simulink model "ideal_source_Motor_DVS_newest_param"  (R2025a)
settings: Solver=daessc  StartTime=0.0  StopTime=2  MaxStep=1e-7  RelTol=1e-3
model workspace (MAT data in the model file):
  FocDiscrTime = 0.0001
  Is_max = 390
  Ld = 0.0002
  Lq = 0.0002
  PolePairs = 13
  Psi = 0.07437
  Rs = 0.06
  compensate_pwm = 0
  piBandwidth = 5000
libraries: fl_lib x18, nesl_utility x15, mcbeeMathTransformLib x7, spsMeanLib x5, slpidlib x5, simulink x2, ee_lib x1, simulink_extras x1
(part 1 of 2)
settings Model: ParameterArgumentNames=FocDiscrTime,PolePairs,Psi  Creator=alexey  LastModifiedBy=alexey
settings SolverCC: ZeroCrossAlgorithm=Adaptive
settings OptimizationCC: DefaultParameterBehavior=Inlined  UseDivisionForNetSlopeComputation=on  GainParamInheritBuiltInType=on  UseFloatMulNetSlope=on  InlineInvariantSignals=on  ReuseModelBlockBuffer=off  EfficientFloat2IntCast=on  LifeSpan=1
settings DebuggingCC: IgnoredZcDiagnostic=none
settings HardwareCC: ProdLongLongMode=on
settings SFSimCC: MATLABDynamicMemAlloc=off
settings RTWCC: GenerateReport=on  LaunchReport=on  GPUComputeCapability=3.5
settings CodeAppCC: ForceParamTrailComments=on
settings GRTTargetCC: RTWCAPISignals=on  RTWCAPIParams=on  CombineSignalStateStructs=on  MatFileLogging=off  SupportVariableSizeSignals=on

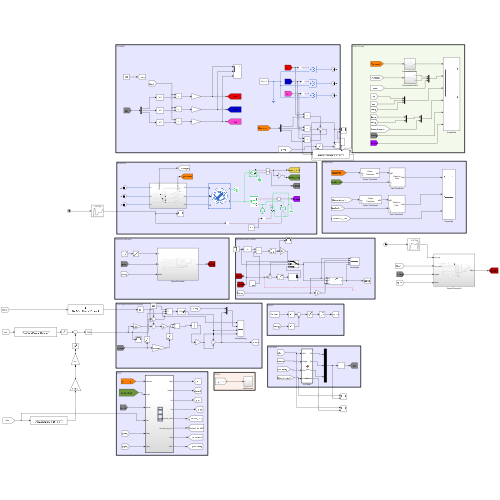
[thumbnail: Simulink's stored preview of the top-level diagram]
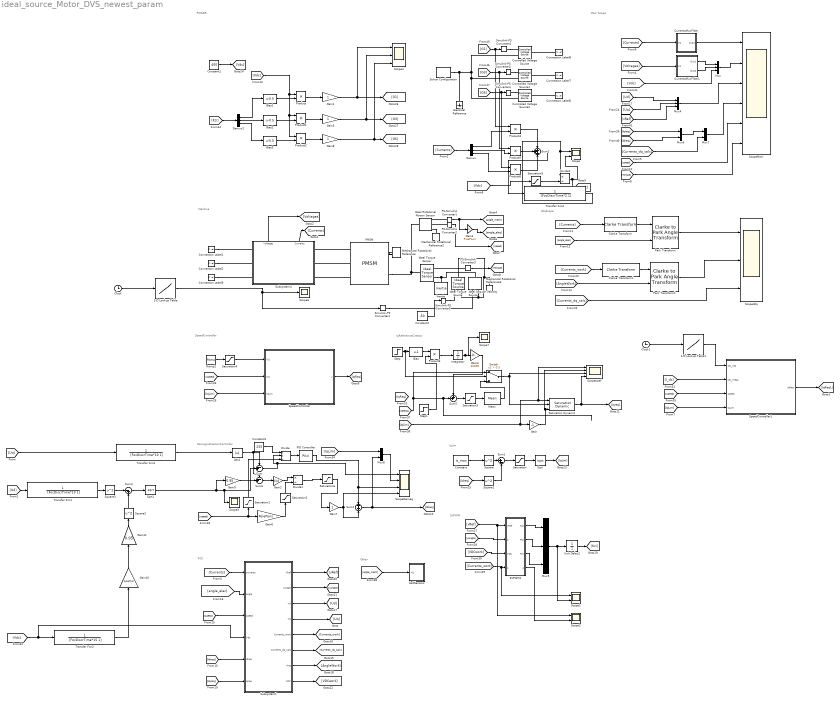
== system ideal_source_Motor_DVS_newest_param ==
  note: Main Scope
  note: POWER
  note: Other
  note: SVPWM
  note: FOC
  note: IqLim
  note: DemagnetizationController
  note: IdIqScope
  note: SpeedController
  note: IqReferenceCreator
  note: Machine
  1-D Lookup Table : Lookup_n-D  NumberOfTableDimensions=1  BreakpointsForDimension1=[0 0.2 0.3 0.45 0.7 1 1.5 1.6 1.7]  Table=[0 270 270 40 40 120 120 220 220]  InternalRulePriority=Speed  RndMeth=Simplest
  1-D Lookup Table1 : Lookup_n-D  NumberOfTableDimensions=1  BreakpointsForDimension1=[0 0.3 1 1.2 1.3 1.4 1.5]  Table=[0 200 150 200 30 250 250]  InternalRulePriority=Speed  RndMeth=Simplest
  Abs1 : Abs  SaturateOnIntegerOverflow=off
  Bias : Bias  Bias=-1  SaturateOnIntegerOverflow=off
  Bias1 : Bias  Bias=-0.5  SaturateOnIntegerOverflow=off
  Bias2 : Bias  Bias=-0.5  SaturateOnIntegerOverflow=off
  Bias3 : Bias  Bias=-0.5  SaturateOnIntegerOverflow=off
  Clarke Transform : mcbeeMathTransformLib/Clarke Transform  VariantControl=Variant2  PowerInvariant=off  UseWithEmbedded=on  PhaseInput=Three inputs
      settings: LibrarySourceBlock=mcbcontrolslib/Clarke Transform
  Clarke Transform1 : mcbeeMathTransformLib/Clarke Transform  VariantControl=Variant2  PowerInvariant=off  UseWithEmbedded=on  PhaseInput=Three inputs
      settings: LibrarySourceBlock=mcbcontrolslib/Clarke Transform
  Clock : Clock
  Clock1 : Clock
  Connection Label1 : ConnectionLabel  Label=A
  Connection Label2 : ConnectionLabel  Label=B
  Connection Label6 : ConnectionLabel  Label=C
  Connection Label7 : ConnectionLabel  Label=B
  Connection Label8 : ConnectionLabel  Label=A
  Connection Label9 : ConnectionLabel  Label=C
  Constant : Constant  Value=Is_max
  Constant1 : Constant  Value=400
  Constant2 : Constant  Value=-50
  Constant3 : Constant  Value=245
  Controlled Voltage Source : fl_lib/Electrical/Electrical Sources/Controlled Voltage Source
  Controlled Voltage Source1 : fl_lib/Electrical/Electrical Sources/Controlled Voltage Source
  Controlled Voltage Source2 : fl_lib/Electrical/Electrical Sources/Controlled Voltage Source
  CurrentsMuxFilter : Subsystem
  CurrentsMuxFilter1 : Subsystem
  Demux : Demux  Outputs=3
  Demux2 : Demux  Outputs=3
  Divide : Product  Inputs=**/
  Divide1 : Product  Inputs=*/
  Divide2 : Product  Inputs=*/
  Electrical Reference : fl_lib/Electrical/Electrical Elements/Electrical Reference
  Gain : Gain  Gain=-1
  Gain{1,5,7..8} (4 alike) : Gain
  Gain10 : Gain  Gain=1/sqrt(3)
  Gain11 : Gain  Gain=0.95
  Gain2 : Gain  Gain=1/Ld
  Gain3 : Gain  Gain=20000
  Gain4 : Gain  Gain=PolePairs
  Gain6 : Gain  Gain=PolePairs
  Gain9 : Gain  Gain=0.95
  HallSensors : Subsystem
  Ideal Angular Velocity Source : fl_lib/Mechanical/Mechanical Sources/Ideal Angular Velocity Source
  Ideal Rotational Motion Sensor : fl_lib/Mechanical/Mechanical Sensors/Ideal Rotational Motion Sensor  reference=foundation.enum.MeasurementReference.difference  acceleration_port=false  velocity_port=true  position_port=true  wrap_angle=false  offset=0 rad
  Ideal Torque Sensor : fl_lib/Mechanical/Mechanical Sensors/Ideal Torque Sensor
  Ideal Torque Source : fl_lib/Mechanical/Mechanical Sources/Ideal Torque Source
  Inertia : fl_lib/Mechanical/Rotational Elements/Inertia  inertia=0.1 kg*m^2  num_ports=foundation.enum.numPorts2.one  w_specify=off  w_priority=High  w=0 rad/s  w_nominal_specify=off  w_nominal_value=1  w_nominal_unit=rad/s  t_specify=off  t_priority=None  t=0 N*m  t_nominal_specify=off  t_nominal_value=1  t_nominal_unit=N*m
  Integrator : Integrator  LimitOutput=on  UpperSaturationLimit=0  LowerSaturationLimit=-2*Is_max/20000
  Mean : spsMeanLib/Mean  Freq=1000  Vinit=0  Ts=0
  Mechanical Rotational Reference : fl_lib/Mechanical/Rotational Elements/Mechanical Rotational Reference
  Mechanical Rotational Reference2 : fl_lib/Mechanical/Rotational Elements/Mechanical Rotational Reference
  Mechanical Rotational Reference3 : fl_lib/Mechanical/Rotational Elements/Mechanical Rotational Reference
  Mux : Mux  Inputs=3
  Mux4 : Mux  Inputs=3
  Mux5 : Mux  Inputs=3
  Mux6 : Mux  Inputs=2
  Mux7 : Mux  Inputs=2
  Mux8 : Mux  Inputs=2
  PID Controller : slpidlib/PID Controller  Controller=PI  Form=Parallel  TimeDomain=Discrete-time  UseExternalTs=off  SampleTime=FocDiscrTime  IntegratorMethod=Forward Euler  FilterMethod=Forward Euler  ControllerParametersSource=internal  P=0.1  I=500  UseKiTs=off  D=0.01  UseExternalDerivativeSource=off  N=100  UseFilter=on  TunerSelectOption=Transfer Function Based (PID Tuner App)  InitialConditionSource=internal  InitialConditionForIntegrator=0  InitialConditionForFilter=0  DifferentiatorICPrevScaledInput=0  ExternalReset=none  TrackingMode=off  Kt=1  LimitOutput=on  SatLimitsSource=internal  UpperSaturationLimit=0  LowerSaturationLimit=-250  LinearizeAsGain=on  AntiWindupMode=clamping  Kb=1  LimitIntegrator=off  UpperIntegratorSaturationLimit=inf  LowerIntegratorSaturationLimit=-inf  POutMin=[]  POutMax=[]  IOutMin=[]  IOutMax=[]  DOutMin=[]  DOutMax=[]  NOutMin=[]  NOutMax=[]  SumOutMin=[]  SumOutMax=[]  SaturationOutMin=[]  SaturationOutMax=[]  PParamMin=[]  PParamMax=[]  IParamMin=[]  IParamMax=[]  DParamMin=[]  DParamMax=[]  NParamMin=[]  NParamMax=[]  KbParamMin=[]  KbParamMax=[]  KtParamMin=[]  KtParamMax=[]  KbOutMin=[]  KbOutMax=[]  KtOutMin=[]  KtOutMax=[]  IntegratorOutMin=[]  IntegratorOutMax=[]  FilterOutMin=[]  FilterOutMax=[]  SumI1OutMin=[]  SumI1OutMax=[]  SumI2OutMin=[]  SumI2OutMax=[]  SumI3OutMin=[]  SumI3OutMax=[]  SumI4OutMin=[]  SumI4OutMax=[]  SumDOutMin=[]  SumDOutMax=[]  DifferentiatorOutMin=[]  DifferentiatorOutMax=[]  FilterDiffOutCoefMin=[]  FilterDiffOutCoefMax=[]  ReciprocalOutMin=[]  ReciprocalOutMax=[]  SumDenOutMin=[]  SumDenOutMax=[]  SumNumOutMin=[]  SumNumOutMax=[]  DivideOutMin=[]  DivideOutMax=[]  UdiffTsProdOutMin=[]  UdiffTsProdOutMax=[]  NTsProdOutMin=[]  NTsProdOutMax=[]  UintegralTsProdOutMin=[]  UintegralTsProdOutMax=[]  UngainTsProdOutMin=[]  UngainTsProdOutMax=[]  ClampingZeroOutDataTypeStr=Inherit: Inherit via back propagation  ClampingZeroOutMin=[]  ClampingZeroOutMax=[]  FilterDenConstantOutDataTypeStr=Inherit: Inherit via back propagation  FilterDenConstantOutMin=[]  FilterDenConstantOutMax=[]  PCopyOutDataTypeStr=Inherit: Inherit via back propagation  PCopyOutMin=[]  PCopyOutMax=[]  NCopyOutDataTypeStr=Inherit: Inherit via back propagation  NCopyOutMin=[]  NCopyOutMax=[]  IntegratorContinuousStateAttributes=''  IntegratorStateMustResolveToSignalObject=off  IntegratorRTWStateStorageClass=Auto  FilterContinuousStateAttributes=''  FilterStateMustResolveToSignalObject=off  FilterRTWStateStorageClass=Auto  ParallelPVariant=InternalParameters  IdealPVariant=Disabled  IVariant=InternalParameters  DVariant=Disabled  IntegratorVariant=Discrete  SatVariant=Enabled  AWVariant=DiscClampingParallel  PCopyVariant=Disabled  TRVariant=Disabled  FdbkBlocksVariant=Forward  IdealPFdbkVariant=Disabled  SatFdbkVariant=Disabled  DerivativeFilterVariant=Disabled  NVariant=Disabled  NCopyVariant=Disabled_SignalSpec  FilterICVariant=Disabled  IntegratorICVariant=InternalICs  ExternalResetVariant=Disabled  TRSumVariant=Passthrough  SumFdbkVariant=Disabled  SumVariant=Sum_PI  TsampFilterVariant=InternalTs  TsampNgainVariant=Passthrough  TsampIntegralVariant=Disabled_SignalSpec  ExternalSaturationOutDataTypeStr=Inherit: Same as second input  DerivativeSourceVariant=Disabled  PreIntVariant=InternalPreInt
  PMSM : ee_lib/Electromechanical/Permanent Magnet/PMSM  port_option=ee.enum.threePhasePort.expanded  winding_type=ee.enum.electromech.statorconfiguration.wye  machine_param=ee.enum.pmsm.parameterization.constant  nPolePairs=PolePairs  pmflux_param=ee.enum.pmflux.fluxlinkage  pm_flux_linkage=Psi Wb  torque_constant=0.074 N*m/A  back_emf_constant=0.06 V*s/rad  stator_param=ee.enum.statorparam.LdLqL0  Ld=Ld H  Lq=Lq H  idVec=[-200, 0, 200] A  iqVec=[-200, 0, 200] A  LdMatrix=0.0002 * ones(3, 3) H  LqMatrix=0.0002 * ones(3, 3) H  PmMatrix=0.1 * ones(3, 3) Wb  ktMatrix=0.18 * ones(3, 3) N*m/A  keMatrix=0.18 * ones(3, 3) V*s/rad  L0=1e-6 uH  Ls=0.0002 H  Lm=-0.00002 H  Ms=0.00002 H  Rs=Rs Ohm  zero_sequence=ee.enum.park.zerosequence.exclude  axes_param=ee.enum.rotorangle.daxis  loss_param=ee.enum.ironloss.none  losses_oc=[0, 0, 0] W  losses_sc=[0, 0, 0] W  f_losses=60 Hz  Isc_losses=95 A  J=0 kg*m^2  lam=0 N*m*s/rad  i_d_specify=on  i_d_priority=High  i_d=0 A  i_d_nominal_specify=off  i_d_nominal_value=1  i_d_nominal_unit=A  i_q_specify=on  i_q_priority=High  i_q=0 A  i_q_nominal_specify=off  i_q_nominal_value=1  i_q_nominal_unit=A  torque_specify=on  torque_priority=High  torque=0 N*m  torque_nominal_specify=off  torque_nominal_value=1  torque_nominal_unit=N*m  angular_velocity_specify=on  angular_velocity_priority=None  angular_velocity=7000 rpm  angular_velocity_nominal_specify=off  angular_velocity_nominal_value=1  angular_velocity_nominal_unit=rpm  angular_position_specify=on  angular_position_priority=High  angular_position=0 deg  angular_position_nominal_specify=off  angular_position_nominal_value=1  angular_position_nominal_unit=deg  alpha=3.93e-3 1/K  alpha_flux=-0.001 1/K  Tmeas=298.15 K  stator_thermal_mass=100 J/K  rotor_thermal_mass=200 J/K  Rm_percent_rotor=90  Rd_percent_rotor=30  temperatureA_specify=off  temperatureA_priority=High  temperatureA=25 degC  temperatureA_nominal_specify=off  temperatureA_nominal_value=1  temperatureA_nominal_unit=degC  temperatureB_specify=off  temperatureB_priority=High  temperatureB=25 degC  temperatureB_nominal_specify=off  temperatureB_nominal_value=1  temperatureB_nominal_unit=degC  temperatureC_specify=off  temperatureC_priority=High  temperatureC=25 degC  temperatureC_nominal_specify=off  temperatureC_nominal_value=1  temperatureC_nominal_unit=degC  temperatureR_specify=off  temperatureR_priority=High  temperatureR=25 degC  temperatureR_nominal_specify=off  temperatureR_nominal_value=1  temperatureR_nominal_unit=degC
      settings: InternalSimscapePortConfiguration="{\"Bottom\":[],\"Left\":[{\"id\":\"a\",\"label\":\"a\",\"type\":\"foundation.electrical.electrical\"},{\"id\":\"b\",\"label\":\"b\",\"type\":\"foundation.electrical.electrical\"},{\"id\":\"c\",\"label\":\"c\",\"type\":\"foundation.electrical.electrical\"}],\"Right\":[{\"id\":\"R\",\"label\":\"R\",\"type\":\"foundation.mechanical.rotational.rotational\"},{\"id\":\"C\",\"label\":\"C\",\"type\":\"foundation.mechanical.rotational.rotational\"}],\"Top\":[]}"
  PS-Simulink Converter1 : nesl_utility/PS-Simulink Converter  PhysicalDomain=network_engine_domain  SubClassName=ps_output  LeftPortType=input  RightPortType=output  PseudoPeriodic=off  Frequencies=[]  VectorFormat=inherit  Unit=inherit  AffineConversion=off
  PS-Simulink Converter2 : nesl_utility/PS-Simulink Converter  PhysicalDomain=network_engine_domain  SubClassName=ps_output  LeftPortType=input  RightPortType=output  PseudoPeriodic=off  Frequencies=[]  VectorFormat=inherit  Unit=inherit  AffineConversion=off
  PS-Simulink Converter3 : nesl_utility/PS-Simulink Converter  PhysicalDomain=network_engine_domain  SubClassName=ps_output  LeftPortType=input  RightPortType=output  PseudoPeriodic=off  Frequencies=[]  VectorFormat=inherit  Unit=inherit  AffineConversion=off
  Park Transform : mcbeeMathTransformLib/Clarke to Park Angle Transform  AxisAlignment=D-axis  UseWithEmbedded=on  PhaseInput=Three inputs  ThetaInput=Electrical position  AngleInput=Radians  N_points=1024
      settings: LibrarySourceBlock=mcbcontrolslib/Park Transform
  Park Transform1 : mcbeeMathTransformLib/Clarke to Park Angle Transform  AxisAlignment=D-axis  UseWithEmbedded=on  PhaseInput=Three inputs  ThetaInput=Electrical position  AngleInput=Radians  N_points=1024
      settings: LibrarySourceBlock=mcbcontrolslib/Park Transform
  Product{,1..6} (7 alike) : Product
  Ramp2 : simulink/Sources/Ramp  slope=300/4e-3  start=1e-3  InitialOutput=0
  SVPWM1 : MATLAB Function  TreatAsAtomicUnit=on  SystemSampleTime=FocDiscrTime/2
  Saturation : Saturate  UpperLimit=inf  LowerLimit=0
  Saturation Dynamic : simulink/Discontinuities/Saturation Dynamic  OutMin=[]  OutMax=[]  OutDataTypeStr=Inherit: Same as second input  OutDataType=fixdt(1, 16)  OutScaling=2^-10  DoSatur=off
  Saturation1 : Saturate  UpperLimit=inf  LowerLimit=1
  Saturation2 : Saturate  UpperLimit=inf  LowerLimit=1
  Saturation3 : Saturate  UpperLimit=inf  LowerLimit=-Is_max
  Saturation4 : Saturate  UpperLimit=600  LowerLimit=0
  Saturation5 : Saturate  UpperLimit=inf  LowerLimit=1
  Saturation6 : Saturate  UpperLimit=0  LowerLimit=-100
  Scope : Scope  NumInputPorts=2
      settings: ActiveDisplayYMinimum=-51831.017888207687  ActiveDisplayYMaximum=5759.0019876081242  DataLoggingVariableName=ScopeData8
  Scope1 : Scope  NumInputPorts=2
      settings: ActiveDisplayYMinimum=-438.55416313604536  ActiveDisplayYMaximum=438.95198817062709
  Scope2 : Scope  NumInputPorts=2
      settings: ActiveDisplayYMinimum=192.19580526011231  ActiveDisplayYMaximum=251.38218785320146  DataLoggingVariableName=ScopeData2
  Scope3 : Scope
      settings: ActiveDisplayYMinimum=58.599899423791321  ActiveDisplayYMaximum=245.7111222862454  DataLoggingVariableName=ScopeData12
  Scope4 : Scope  NumInputPorts=3
      settings: ActiveDisplayYMinimum=-300  ActiveDisplayYMaximum=-100  DataLoggingVariableName=ScopeData14
  Scope6 : Scope
      settings: ActiveDisplayYMinimum=-68.247393749999986  ActiveDisplayYMaximum=614.22654375  DataLoggingVariableName=ScopeData15
  Scope7 : Scope
      settings: DataLoggingVariableName=ScopeData16
  ScopeDemag : Scope  NumInputPorts=4
      settings: ActiveDisplayYMinimum=100.15963791243919  ActiveDisplayYMaximum=100.26275452875461  DataLoggingVariableName=ScopeData7
  ScopeIdIq : Scope  NumInputPorts=3
      settings: ActiveDisplayYMinimum=-200.18878641188479  ActiveDisplayYMaximum=389.61354814376449  DataLoggingVariableName=ScopeData13
  ScopeIqref : Scope  NumInputPorts=4
      settings: ActiveDisplayYMinimum=300.59489839356036  ActiveDisplayYMaximum=316.60056684515996  DataLoggingVariableName=ScopeData11
  ScopeMain : Scope  NumInputPorts=6
      settings: ActiveDisplayYMinimum=-484.90618085327424  ActiveDisplayYMaximum=498.32290898369712  DataLoggingVariableName=ScopeData9
  Simulink-PS Converter1 : nesl_utility/Simulink-PS Converter  PhysicalDomain=network_engine_domain  SubClassName=ps_input  LeftPortType=input  RightPortType=output  PseudoPeriodic=off  Frequencies=[]  NoiseDistribution=none  NoiseParameters=[]  Unit=1  AffineConversion=off  FilteringAndDerivatives=filter  SimscapeFilterOrder=1  InputFilterTimeConstant=1e-3  UdotUserProvided=0
  Simulink-PS Converter2 : nesl_utility/Simulink-PS Converter  PhysicalDomain=network_engine_domain  SubClassName=ps_input  LeftPortType=input  RightPortType=output  PseudoPeriodic=off  Frequencies=[]  NoiseDistribution=none  NoiseParameters=[]  Unit=1  AffineConversion=off  FilteringAndDerivatives=provide  SimscapeFilterOrder=1  InputFilterTimeConstant=0.001  UdotUserProvided=0
  Simulink-PS Converter3 : nesl_utility/Simulink-PS Converter  PhysicalDomain=network_engine_domain  SubClassName=ps_input  LeftPortType=input  RightPortType=output  PseudoPeriodic=off  Frequencies=[]  NoiseDistribution=none  NoiseParameters=[]  Unit=1  AffineConversion=off  FilteringAndDerivatives=provide  SimscapeFilterOrder=1  InputFilterTimeConstant=0.001  UdotUserProvided=0
  Simulink-PS Converter4 : nesl_utility/Simulink-PS Converter  PhysicalDomain=network_engine_domain  SubClassName=ps_input  LeftPortType=input  RightPortType=output  PseudoPeriodic=off  Frequencies=[]  NoiseDistribution=none  NoiseParameters=[]  Unit=1  AffineConversion=off  FilteringAndDerivatives=provide  SimscapeFilterOrder=1  InputFilterTimeConstant=0.001  UdotUserProvided=0
  Simulink-PS Converter5 : nesl_utility/Simulink-PS Converter  PhysicalDomain=network_engine_domain  SubClassName=ps_input  LeftPortType=input  RightPortType=output  PseudoPeriodic=off  Frequencies=[]  NoiseDistribution=none  NoiseParameters=[]  Unit=1  AffineConversion=off  FilteringAndDerivatives=filter  SimscapeFilterOrder=1  InputFilterTimeConstant=1e-3  UdotUserProvided=0
  Solver Configuration : nesl_utility/Solver Configuration  PhysicalDomain=network_engine_domain  SubClassName=solver  LeftPortType=input  RightPortType=generic  Tones=[]  Harmonics=[]  SimulateNoise=off  Profile=off  UseLocalSampling=off  EnableSwitchedLinearOptims=on  FrequencyDomain=off  UseCCode=off  RelTol=0.001  AbsTol=0.001  MinStep=1e-09  ToWorkspace=off  RevertToSquareIcSolve=off  NumHomotopyIterations=100  PhasorMode=off  PhasorModeNumHarmonics=1  ConsistencySolver=NEWTON_XTOL_AFTER_FTOL  IndexReductionMethod=DerivativeReplacement  DoDC=off  ResidualTolerance=1e-09  ConsistencyTolSource=GLOBAL  ConsistencyAbsTol=0.001  ConsistencyRelTol=0.001  ConsistencyTolFactor=0.001  UseLocalSolver=off  LocalSolverChoice=NE_BACKWARD_EULER_ADVANCER  ResolveIndetEquations=on  FunctionEvalNumThread=1  LocalSolverSampleTime=0.001  DoFixedCost=off  MaxNonlinIter=3  MaxModeIter=2  ComputeImpulses=off  ImpulseIterations=2  LinearAlgebra=auto  LinearAlgebraNumThread=0  EquationFormulation=NE_TIME_EF  DelaysMemoryBudget=1024  AutomaticFiltering=on  FilteringTimeConstant=0.001  PartitionStorageMethod=AS_NEEDED  PartitionMemoryBudget=1024  PartitionMethod=ROBUST  MultibodyUseLocalSolver=off  MultibodyLocalSolverChoice=ODE1  MultibodyLocalSolverSampleTime=0.001
  SpeedController : Subsystem
  SpeedController1 : Subsystem
  Sqrt : Sqrt
  Sqrt1 : Sqrt
  Square{,1..3} (4 alike) : Math  Operator=square
  Step : Step  Time=2  Before=1  After=0  SampleTime=0
  Step1 : Step  Time=0.7  Before=1  After=-1  SampleTime=0
  Subsystem1 : Subsystem  TreatAsAtomicUnit=on  SystemSampleTime=FocDiscrTime
  Subsystem4 : Subsystem
      settings: PortSchema="{\"entries\":[{\"content\":{\"sides\":[{\"content\":{},\"type\":\"ConnectorPlacement.EquallySpacedRectSide\",\"uuid\":\"18ff9a98-da5f-4d42-bf88-8b80acaefaab\"},{\"content\":{\"connectorIds\":[\"Out1\",\"Out2\"],\"side\":\"RIGHT\"},\"type\":\"ConnectorPlacement.EquallySpacedRectSide\",\"uuid\":\"2ae2e449-c022-4e43-8d74-e7903f555369\"},{\"content\":{\"connectorIds\":[\"LConn1\",\"LConn2\",\"LConn3\"],\"side\":\"TOP\"},\"type\":\"ConnectorPlacement.EquallySpacedRectSide\",\"uuid\":\"55b123c9-903d-428f-ba92-02a5913ccae5\"},{\"content\":{\"connectorIds\":[\"RConn1\",\"RConn2\",\"RConn3\"],\"side\":\"BOTTOM\"},\"type\":\"ConnectorPlacement.EquallySpacedRectSide\",\"uuid\":\"b028b0af-4fd3-4535-8d3b-f50dc0cabb29\"}]},\"type\":\"ConnectorPlacement.EquallySpacedConnector\",\"uuid\":\"08d0fd08-360e-4301-974e-a78b2c2bf0b9\"}],\"packageUris\":[\"http://schema.mathworks.com/mf0/Connector/R2020b\"],\"version\":\"1.0\"}"
  Sum : Sum  Inputs=-+|
  Sum1 : Sum  Inputs=|+-
  Sum2 : Sum  Inputs=+++
  Sum3 : Sum  Inputs=|-+
  Sum4 : Sum
  Sum5 : Sum  Inputs=++|
  Sum6 : Sum  Inputs=-+|
  Switch : Switch  Criteria=u2 > Threshold  Threshold=0.5  SaturateOnIntegerOverflow=off  InputSameDT=off
  Transfer Fcn1 : TransferFcn  Denominator=[FocDiscrTime*10 1]
  Transfer Fcn2 : TransferFcn  Denominator=[FocDiscrTime*15 1]
  Transfer Fcn3 : TransferFcn  Denominator=[FocDiscrTime*10 1]
  Transfer Fcn4 : TransferFcn  Denominator=[FocDiscrTime*2 1]
  Unit Delay2 : UnitDelay  SampleTime=FocDiscrTime/2  HasFrameUpgradeWarning=on
  wires:
  CurrentsMuxFilter/1(Out2) -> ScopeMain/1
  [Currents] -> CurrentsMuxFilter/1(In1)
  Mux/1 -> ScopeMain/2
  CurrentsMuxFilter1/1(Out1) -> Mux/1
  [Torque] -> ScopeMain/6
  [speed] -> ScopeMain/5
  [Vdc] -> Mux/3
  CurrentsMuxFilter1/2(Out2) -> Mux/2
  [Voltages] -> CurrentsMuxFilter1/1(In1)
  [Ud] -> Mux4/1
  [Uq] -> Mux4/2
  Mux4/1 -> ScopeMain/3
  [Currents_dq_calc] -> Mux7/2
  [Idreq] -> Mux6/2
  [Iqreq] -> Mux6/1
  Mux6/1 -> Mux7/1
  Mux7/1 -> ScopeMain/4
  [vRef] -> Mux4/3
  Gain8/1 -> [G5], Scope4/3
  Gain5/1 -> [G3], Scope4/2
  Gain1/1 -> [G1], Scope4/1
  [Vdc] -> Product/1, Product1/1, Product2/1
  Product2/1 -> Gain8/1
  Product1/1 -> Gain5/1
  Product/1 -> Gain1/1
  Bias3/1 -> Product2/2
  Bias2/1 -> Product1/2
  Bias1/1 -> Product/2
  [G3] -> Product5/1, Simulink-PS Converter3/1
  [G5] -> Product6/1, Simulink-PS Converter4/1
  [G1] -> Product4/1, Simulink-PS Converter2/1
  Demux2/3 -> Bias3/1
  Demux2/2 -> Bias2/1
  Demux2/1 -> Bias1/1
  [Kzi] -> Demux2/1
  Saturation1/1 -> Divide/3
  Constant3/1 -> Divide/1
  Divide/1 -> PID Controller/1
  Gain11/1 -> Square2/1
  Saturation6/1 -> Gain7/1
  Gain2/1 -> Divide1/1
  Transfer Fcn3/1 -> Abs1/1
  Divide1/1 -> Saturation6/1
  Gain9/1 -> Sum6/2
  Gain7/1 -> ScopeDemag/4, Sum4/2
  Sum6/1 -> Gain2/1
  Mux8/1 -> ScopeDemag/2
  Transfer Fcn2/1 -> Gain10/1
  Abs1/1 -> Sum/1, Sum6/1
  Sum/1 -> ScopeDemag/1, Divide/2
  Clock/1 -> 1-D Lookup Table/1
  Constant2/1 -> Simulink-PS Converter5/1
  [Idreq] -> Square1/1
  [IqReq1] -> Switch/1, Sum5/2
  Saturation3/1 -> Mean/1
  Gain3/1 -> Sum5/1
  Sum5/1 -> Saturation3/1
  Mean/1 -> Switch/3
  Integrator/1 -> Gain3/1, Scope7/1
  Product3/1 -> Integrator/1
  Saturation Dynamic/1 -> [Iqreq], ScopeIqref/4
  Switch/1 -> Saturation Dynamic/2, ScopeIqref/3
  [IqLim] -> Gain/1, ScopeIqref/1, Saturation Dynamic/1
  Gain/1 -> ScopeIqref/2, Saturation Dynamic/3
  Step1/1 -> Product3/2
  Step/1 -> Switch/2, Bias/1
  Bias/1 -> Product3/1
  1-D Lookup Table/1 -> Scope6/1, Simulink-PS Converter1/1
  [Ud] -> Transfer Fcn1/1
  Sum3/1 -> Sqrt1/1
  Square3/1 -> Sum3/1
  Transfer Fcn1/1 -> Square3/1
  Gain10/1 -> Gain11/1
  Square2/1 -> Sum3/2
  Sqrt1/1 -> Sum/2, Scope3/1, Gain9/1
  SVPWM1/4(vRefwork) -> Scope2/2
  [Uq] -> Transfer Fcn3/1
  [angle_mech] -> HallSensors/1(In1)
  PID Controller/1 -> ScopeDemag/3, Sum4/1
  Gain6/1 -> Saturation2/1
  [IqLim] -> Mux8/1
  [IqLim] -> SpeedController/3(IqLim)
  SVPWM1/3(Tct) -> Mux5/3
  SVPWM1/2(Tbt) -> Mux5/2
  SVPWM1/1(Tat) -> Mux5/1
  [VDCwork] -> SVPWM1/3(VDC)
  [vAngle] -> SVPWM1/2(vAngle)
  [Currents_work] -> SVPWM1/4(Currents), Scope1/1
  [vRef] -> SVPWM1/1(vRef), Scope2/1
  Subsystem1/1(vRef) -> [vRef]
  Subsystem1/8(VDC) -> [VDCwork]
  Subsystem1/2(vAngle) -> [vAngle]
  Unit Delay2/1 -> [Kzi]
  Mux5/1 -> Unit Delay2/1, Scope1/2
  Subsystem1/7(Ang) -> [AngleWork]
  Subsystem1/3(Vd) -> [Ud]
  [Currents_work] -> Clarke Transform1/1
  Clarke Transform1/1 -> Park Transform1/1
  [AngleWork] -> Park Transform1/2
  Park Transform1/1 -> ScopeIdIq/2
  Subsystem1/6(Currents_dq_calc) -> [Currents_dq_calc]
  Subsystem1/5(Currents_work) -> [Currents_work]
  Saturation4/1 -> SpeedController/1(In1)
  [Iqreq] -> Subsystem1/6(Iqreq)
  [Idreq] -> Subsystem1/5(Idreq)
  Subsystem1/4(Vq) -> [Uq]
  SpeedController/1(y) -> [IqReq]
  [speed] -> SpeedController/2(In2)
  Ramp2/1 -> Saturation4/1
  [speed] -> Gain6/1, Saturation1/1
  [Currents_dq_calc] -> ScopeIdIq/3
  Park Transform/1 -> ScopeIdIq/1
  [angle_elec] -> Park Transform/2
  Clarke Transform/1 -> Park Transform/1
  [Currents] -> Clarke Transform/1
  PS-Simulink Converter1/1 -> [angle_mech], Gain4/1
  Gain4/1 -> [angle_elec]
  [speed] -> Subsystem1/3(speed)
  Subsystem4/2(Currents) -> [Currents]
  Square1/1 -> Sum1/2
  Sum4/1 -> Mux8/2, [Idreq]
  Square/1 -> Sum1/1
  PS-Simulink Converter2/1 -> [speed]
  [Currents] -> Subsystem1/1(currents)
  Sum1/1 -> Saturation/1
  Saturation/1 -> Sqrt/1
  PS-Simulink Converter3/1 -> [Torque]
  Sqrt/1 -> [IqLim]
  Constant/1 -> Square/1
  Subsystem4/1(Voltages) -> [Voltages]
  [angle_elec] -> Subsystem1/2(angle)
  Saturation2/1 -> Divide1/2
  Constant1/1 -> [Vdc]
  [Vdc] -> Subsystem1/4(Vdc), Transfer Fcn2/1
  [Currents] -> Demux/1
  Demux/1 -> Product4/2
  Demux/2 -> Product5/2
  Demux/3 -> Product6/2
  Product4/1 -> Sum2/1
  Product5/1 -> Sum2/2
  Product6/1 -> Sum2/3
  Sum2/1 -> Transfer Fcn4/1
  [Vdc] -> Saturation5/1
  Divide2/1 -> [I_dc], Scope/2
  Saturation5/1 -> Divide2/2
  Transfer Fcn4/1 -> Divide2/1, Scope/1
  Clock1/1 -> 1-D Lookup Table1/1
  [speed] -> SpeedController1/3(speed)
  SpeedController1/1(IqReq) -> [IqReq1]
  [I_dc] -> SpeedController1/2(Idc_meas)
  1-D Lookup Table1/1 -> SpeedController1/1(Idc_req)
  [IqLim] -> SpeedController1/4(IqLim)
  connections:
  Solver Configuration/RConn1 -- Electrical Reference/LConn1 -- Controlled Voltage Source/RConn2 -- Controlled Voltage Source2/RConn2 -- Controlled Voltage Source1/RConn2
  Simulink-PS Converter3/RConn1 -- Controlled Voltage Source1/RConn1
  Connection Label7/LConn1 -- Controlled Voltage Source1/LConn1
  Simulink-PS Converter2/RConn1 -- Controlled Voltage Source/RConn1
  Connection Label8/LConn1 -- Controlled Voltage Source/LConn1
  Connection Label6/LConn1 -- Controlled Voltage Source2/LConn1
  Simulink-PS Converter4/RConn1 -- Controlled Voltage Source2/RConn1
  Ideal Torque Sensor/LConn1 -- Ideal Rotational Motion Sensor/LConn1 -- PMSM/RConn1
  Mechanical Rotational Reference3/LConn1 -- Ideal Torque Source/RConn2 -- Ideal Angular Velocity Source/RConn2 -- Ideal Torque Source/LConn1
  Ideal Torque Sensor/RConn1 -- Inertia/LConn1 -- Ideal Angular Velocity Source/LConn1
  PS-Simulink Converter2/LConn1 -- Ideal Rotational Motion Sensor/RConn2
  PMSM/RConn2 -- Mechanical Rotational Reference/LConn1
  Connection Label1/LConn1 -- Subsystem4/LConn3
  PMSM/LConn2 -- Subsystem4/RConn2
  PS-Simulink Converter3/LConn1 -- Ideal Torque Sensor/RConn2
  Simulink-PS Converter1/RConn1 -- Ideal Angular Velocity Source/RConn1
  Connection Label9/LConn1 -- Subsystem4/LConn1
  Connection Label2/LConn1 -- Subsystem4/LConn2
  PMSM/LConn3 -- Subsystem4/RConn3
  PS-Simulink Converter1/LConn1 -- Ideal Rotational Motion Sensor/RConn3
  PMSM/LConn1 -- Subsystem4/RConn1
  Ideal Rotational Motion Sensor/RConn1 -- Mechanical Rotational Reference2/LConn1
  Simulink-PS Converter5/RConn1 -- Ideal Torque Source/RConn1

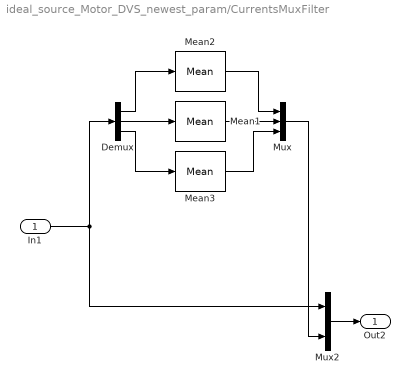
== system ideal_source_Motor_DVS_newest_param/CurrentsMuxFilter ==
  In1 : Inport
  Demux : Demux  Outputs=3
  Mean1 : spsMeanLib/Mean  Freq=20000  Vinit=0  Ts=0
  Mean2 : spsMeanLib/Mean  Freq=20000  Vinit=0  Ts=0
  Mean3 : spsMeanLib/Mean  Freq=20000  Vinit=0  Ts=0
  Mux : Mux  Inputs=3
  Mux2 : Mux  Inputs=2
  Out2 : Outport
  wires:
  Mean3/1 -> Mux/3
  Mean1/1 -> Mux/2
  Mean2/1 -> Mux/1
  Demux/3 -> Mean3/1
  Demux/2 -> Mean1/1
  Demux/1 -> Mean2/1
  Mux2/1 -> Out2/1
  In1/1 -> Mux2/1, Demux/1
  Mux/1 -> Mux2/2

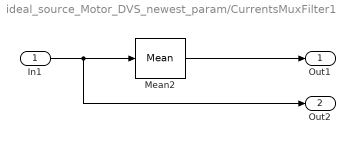
== system ideal_source_Motor_DVS_newest_param/CurrentsMuxFilter1 ==
  In1 : Inport
  Mean2 : spsMeanLib/Mean  Freq=20000  Vinit=0  Ts=0
  Out1 : Outport
  Out2 : Outport  Port=2
  wires:
  In1/1 -> Mean2/1, Out2/1
  Mean2/1 -> Out1/1

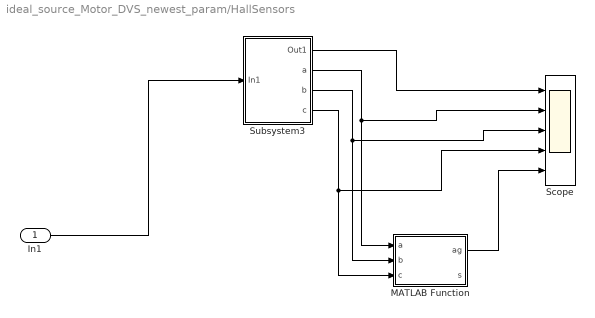
== system ideal_source_Motor_DVS_newest_param/HallSensors ==
  In1 : Inport
  MATLAB Function : MATLAB Function  TreatAsAtomicUnit=on  SystemSampleTime=1/40000
  Scope : Scope  NumInputPorts=5
      settings: ActiveDisplayYMinimum=-0.7854  ActiveDisplayYMaximum=7.06858  DataLoggingVariableName=ScopeData3
  Subsystem3 : Subsystem
  wires:
  Subsystem3/1(Out1) -> Scope/1
  Subsystem3/4(c) -> Scope/4, MATLAB Function/3(c)
  Subsystem3/2("a ") -> Scope/2, MATLAB Function/1(a)
  MATLAB Function/1(ag) -> Scope/5
  Subsystem3/3(b) -> Scope/3, MATLAB Function/2(b)
  In1/1 -> Subsystem3/1(In1)

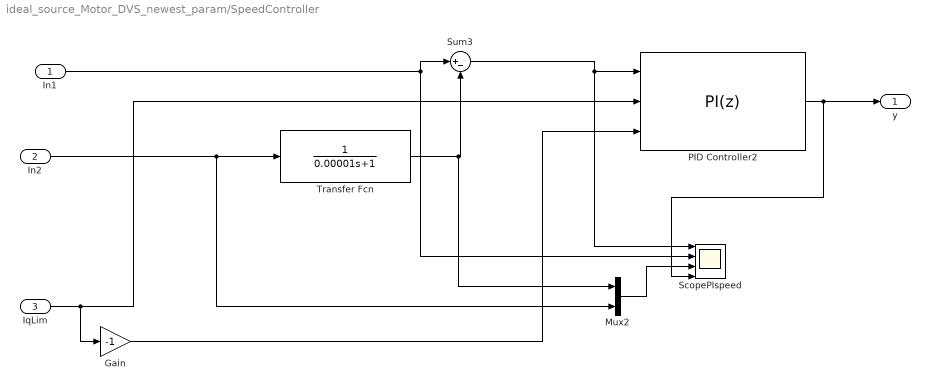
== system ideal_source_Motor_DVS_newest_param/SpeedController ==
  In1 : Inport
  In2 : Inport  Port=2
  IqLim : Inport  Port=3
  Gain : Gain  Gain=-1
  Mux2 : Mux  Inputs=2
  PID Controller2 : slpidlib/PID Controller  Controller=PI  Form=Parallel  TimeDomain=Discrete-time  UseExternalTs=off  SampleTime=FocDiscrTime  IntegratorMethod=Forward Euler  FilterMethod=Forward Euler  ControllerParametersSource=internal  P=5  I=1  UseKiTs=off  D=0  UseExternalDerivativeSource=off  N=100  UseFilter=on  TunerSelectOption=Transfer Function Based (PID Tuner App)  InitialConditionSource=internal  InitialConditionForIntegrator=0  InitialConditionForFilter=0  DifferentiatorICPrevScaledInput=0  ExternalReset=none  TrackingMode=off  Kt=1  LimitOutput=on  SatLimitsSource=external  UpperSaturationLimit=350  LowerSaturationLimit=-3  LinearizeAsGain=on  AntiWindupMode=clamping  Kb=1  LimitIntegrator=off  UpperIntegratorSaturationLimit=inf  LowerIntegratorSaturationLimit=-inf  POutMin=[]  POutMax=[]  IOutMin=[]  IOutMax=[]  DOutMin=[]  DOutMax=[]  NOutMin=[]  NOutMax=[]  SumOutMin=[]  SumOutMax=[]  SaturationOutMin=[]  SaturationOutMax=[]  PParamMin=[]  PParamMax=[]  IParamMin=[]  IParamMax=[]  DParamMin=[]  DParamMax=[]  NParamMin=[]  NParamMax=[]  KbParamMin=[]  KbParamMax=[]  KtParamMin=[]  KtParamMax=[]  KbOutMin=[]  KbOutMax=[]  KtOutMin=[]  KtOutMax=[]  IntegratorOutMin=[]  IntegratorOutMax=[]  FilterOutMin=[]  FilterOutMax=[]  SumI1OutMin=[]  SumI1OutMax=[]  SumI2OutMin=[]  SumI2OutMax=[]  SumI3OutMin=[]  SumI3OutMax=[]  SumI4OutMin=[]  SumI4OutMax=[]  SumDOutMin=[]  SumDOutMax=[]  DifferentiatorOutMin=[]  DifferentiatorOutMax=[]  FilterDiffOutCoefMin=[]  FilterDiffOutCoefMax=[]  ReciprocalOutMin=[]  ReciprocalOutMax=[]  SumDenOutMin=[]  SumDenOutMax=[]  SumNumOutMin=[]  SumNumOutMax=[]  DivideOutMin=[]  DivideOutMax=[]  UdiffTsProdOutMin=[]  UdiffTsProdOutMax=[]  NTsProdOutMin=[]  NTsProdOutMax=[]  UintegralTsProdOutMin=[]  UintegralTsProdOutMax=[]  UngainTsProdOutMin=[]  UngainTsProdOutMax=[]  ClampingZeroOutDataTypeStr=Inherit: Inherit via back propagation  ClampingZeroOutMin=[]  ClampingZeroOutMax=[]  FilterDenConstantOutDataTypeStr=Inherit: Inherit via back propagation  FilterDenConstantOutMin=[]  FilterDenConstantOutMax=[]  PCopyOutDataTypeStr=Inherit: Inherit via back propagation  PCopyOutMin=[]  PCopyOutMax=[]  NCopyOutDataTypeStr=Inherit: Inherit via back propagation  NCopyOutMin=[]  NCopyOutMax=[]  IntegratorContinuousStateAttributes=''  IntegratorStateMustResolveToSignalObject=off  IntegratorRTWStateStorageClass=Auto  FilterContinuousStateAttributes=''  FilterStateMustResolveToSignalObject=off  FilterRTWStateStorageClass=Auto  ParallelPVariant=InternalParameters  IdealPVariant=Disabled  IVariant=InternalParameters  DVariant=Disabled  IntegratorVariant=Discrete  SatVariant=External  AWVariant=DiscClampingParallel  PCopyVariant=Disabled  TRVariant=Disabled  FdbkBlocksVariant=Forward  IdealPFdbkVariant=Disabled  SatFdbkVariant=Disabled  DerivativeFilterVariant=Disabled  NVariant=Disabled  NCopyVariant=Disabled_SignalSpec  FilterICVariant=Disabled  IntegratorICVariant=InternalICs  ExternalResetVariant=Disabled  TRSumVariant=Passthrough  SumFdbkVariant=Disabled  SumVariant=Sum_PI  TsampFilterVariant=InternalTs  TsampNgainVariant=Passthrough  TsampIntegralVariant=Disabled_SignalSpec  ExternalSaturationOutDataTypeStr=Inherit: Same as second input  DerivativeSourceVariant=Disabled  PreIntVariant=InternalPreInt
  ScopePIspeed : Scope  NumInputPorts=4
      settings: ActiveDisplayYMinimum=-74.200839679499552  ActiveDisplayYMaximum=662.92601742403372  DataLoggingVariableName=ScopeData10
  Sum3 : Sum  Inputs=|+-
  Transfer Fcn : TransferFcn  Denominator=[0.00001 1]
  y : Outport
  wires:
  Gain/1 -> PID Controller2/3
  IqLim/1 -> PID Controller2/2, Gain/1
  In1/1 -> ScopePIspeed/2, Sum3/1
  Transfer Fcn/1 -> Sum3/2, Mux2/1
  Sum3/1 -> PID Controller2/1, ScopePIspeed/1
  PID Controller2/1 -> ScopePIspeed/4, y/1
  In2/1 -> Transfer Fcn/1, Mux2/2
  Mux2/1 -> ScopePIspeed/3

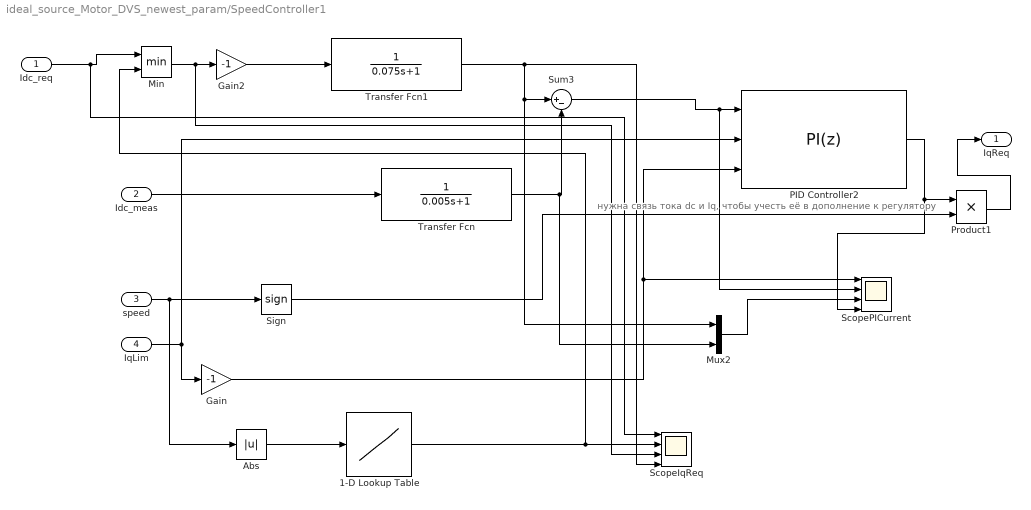
== system ideal_source_Motor_DVS_newest_param/SpeedController1 ==
  note: нужна связь тока dc и Iq, чтобы учесть её в дополнение к регулятору
  Idc_req : Inport
  Idc_meas : Inport  Port=2
  speed : Inport  Port=3
  IqLim : Inport  Port=4
  1-D Lookup Table : Lookup_n-D  NumberOfTableDimensions=1  BreakpointsForDimension1=[0 550 600 1200 1925 2350 2400 2450]*0.1047  Table=[0 0 69 115 115 50 0 0]  InternalRulePriority=Speed  RndMeth=Simplest
  Abs : Abs  SaturateOnIntegerOverflow=off
  Gain : Gain  Gain=-1
  Gain2 : Gain  Gain=-1
  Min : MinMax  Inputs=2
  Mux2 : Mux  Inputs=2
  PID Controller2 : slpidlib/PID Controller  Controller=PI  Form=Parallel  TimeDomain=Discrete-time  UseExternalTs=off  SampleTime=FocDiscrTime  IntegratorMethod=Forward Euler  FilterMethod=Forward Euler  ControllerParametersSource=internal  P=5  I=450  UseKiTs=off  D=0  UseExternalDerivativeSource=off  N=100  UseFilter=on  TunerSelectOption=Transfer Function Based (PID Tuner App)  InitialConditionSource=internal  InitialConditionForIntegrator=0  InitialConditionForFilter=0  DifferentiatorICPrevScaledInput=0  ExternalReset=none  TrackingMode=off  Kt=1  LimitOutput=on  SatLimitsSource=external  UpperSaturationLimit=350  LowerSaturationLimit=-3  LinearizeAsGain=on  AntiWindupMode=clamping  Kb=1  LimitIntegrator=off  UpperIntegratorSaturationLimit=inf  LowerIntegratorSaturationLimit=-inf  POutMin=[]  POutMax=[]  IOutMin=[]  IOutMax=[]  DOutMin=[]  DOutMax=[]  NOutMin=[]  NOutMax=[]  SumOutMin=[]  SumOutMax=[]  SaturationOutMin=[]  SaturationOutMax=[]  PParamMin=[]  PParamMax=[]  IParamMin=[]  IParamMax=[]  DParamMin=[]  DParamMax=[]  NParamMin=[]  NParamMax=[]  KbParamMin=[]  KbParamMax=[]  KtParamMin=[]  KtParamMax=[]  KbOutMin=[]  KbOutMax=[]  KtOutMin=[]  KtOutMax=[]  IntegratorOutMin=[]  IntegratorOutMax=[]  FilterOutMin=[]  FilterOutMax=[]  SumI1OutMin=[]  SumI1OutMax=[]  SumI2OutMin=[]  SumI2OutMax=[]  SumI3OutMin=[]  SumI3OutMax=[]  SumI4OutMin=[]  SumI4OutMax=[]  SumDOutMin=[]  SumDOutMax=[]  DifferentiatorOutMin=[]  DifferentiatorOutMax=[]  FilterDiffOutCoefMin=[]  FilterDiffOutCoefMax=[]  ReciprocalOutMin=[]  ReciprocalOutMax=[]  SumDenOutMin=[]  SumDenOutMax=[]  SumNumOutMin=[]  SumNumOutMax=[]  DivideOutMin=[]  DivideOutMax=[]  UdiffTsProdOutMin=[]  UdiffTsProdOutMax=[]  NTsProdOutMin=[]  NTsProdOutMax=[]  UintegralTsProdOutMin=[]  UintegralTsProdOutMax=[]  UngainTsProdOutMin=[]  UngainTsProdOutMax=[]  ClampingZeroOutDataTypeStr=Inherit: Inherit via back propagation  ClampingZeroOutMin=[]  ClampingZeroOutMax=[]  FilterDenConstantOutDataTypeStr=Inherit: Inherit via back propagation  FilterDenConstantOutMin=[]  FilterDenConstantOutMax=[]  PCopyOutDataTypeStr=Inherit: Inherit via back propagation  PCopyOutMin=[]  PCopyOutMax=[]  NCopyOutDataTypeStr=Inherit: Inherit via back propagation  NCopyOutMin=[]  NCopyOutMax=[]  IntegratorContinuousStateAttributes=''  IntegratorStateMustResolveToSignalObject=off  IntegratorRTWStateStorageClass=Auto  FilterContinuousStateAttributes=''  FilterStateMustResolveToSignalObject=off  FilterRTWStateStorageClass=Auto  ParallelPVariant=InternalParameters  IdealPVariant=Disabled  IVariant=InternalParameters  DVariant=Disabled  IntegratorVariant=Discrete  SatVariant=External  AWVariant=DiscClampingParallel  PCopyVariant=Disabled  TRVariant=Disabled  FdbkBlocksVariant=Forward  IdealPFdbkVariant=Disabled  SatFdbkVariant=Disabled  DerivativeFilterVariant=Disabled  NVariant=Disabled  NCopyVariant=Disabled_SignalSpec  FilterICVariant=Disabled  IntegratorICVariant=InternalICs  ExternalResetVariant=Disabled  TRSumVariant=Passthrough  SumFdbkVariant=Disabled  SumVariant=Sum_PI  TsampFilterVariant=InternalTs  TsampNgainVariant=Passthrough  TsampIntegralVariant=Disabled_SignalSpec  ExternalSaturationOutDataTypeStr=Inherit: Same as second input  DerivativeSourceVariant=Disabled  PreIntVariant=InternalPreInt
  Product1 : Product
  ScopeIqReq : Scope  NumInputPorts=4
      settings: ActiveDisplayYMinimum=-31.249999999999993  ActiveDisplayYMaximum=281.25  DataLoggingVariableName=ScopeData14
  ScopePICurrent : Scope  NumInputPorts=4
      settings: ActiveDisplayYMinimum=-315.28897228681205  ActiveDisplayYMaximum=-312.39924941869185  DataLoggingVariableName=ScopeData10
  Sign : Signum
  Sum3 : Sum  Inputs=|+-
  Transfer Fcn : TransferFcn  Denominator=[0.005 1]
  Transfer Fcn1 : TransferFcn  Denominator=[0.075 1]
  IqReq : Outport
  wires:
  Transfer Fcn1/1 -> Sum3/1, Mux2/1, ScopeIqReq/4
  Idc_req/1 -> Min/1, ScopeIqReq/1
  Gain/1 -> ScopePICurrent/1, PID Controller2/3
  IqLim/1 -> Gain/1, PID Controller2/2
  1-D Lookup Table/1 -> ScopeIqReq/2, Min/2
  Abs/1 -> 1-D Lookup Table/1
  Product1/1 -> IqReq/1
  Idc_meas/1 -> Transfer Fcn/1
  Min/1 -> Gain2/1, ScopeIqReq/3
  Sign/1 -> Product1/2
  speed/1 -> Sign/1, Abs/1
  Mux2/1 -> ScopePICurrent/3
  PID Controller2/1 -> ScopePICurrent/4, Product1/1
  Sum3/1 -> PID Controller2/1, ScopePICurrent/2
  Transfer Fcn/1 -> Sum3/2, Mux2/2
  Gain2/1 -> Transfer Fcn1/1

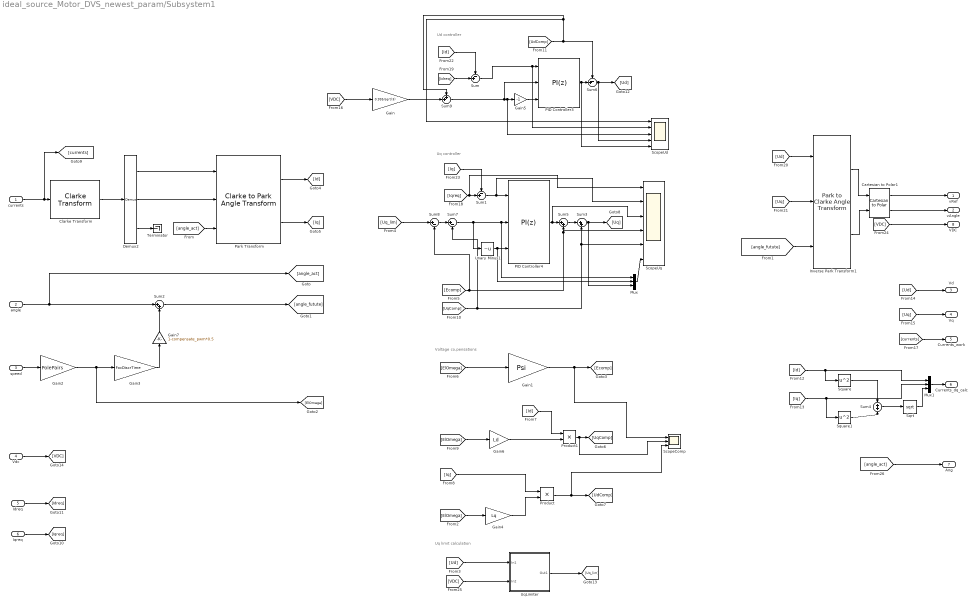
== system ideal_source_Motor_DVS_newest_param/Subsystem1 ==
  note: Uq controller
  note: Ud controller
  note: Voltage co,pensations
  note: Uq limit calculation
  currents : Inport
  angle : Inport  Port=2
  speed : Inport  Port=3
  Vdc : Inport  Port=4
  Idreq : Inport  Port=5
  Iqreq : Inport  Port=6
  Cartesian to Polar1 : simulink_extras/Transformations/Cartesian to Polar
  Clarke Transform : mcbeeMathTransformLib/Clarke Transform  VariantControl=Variant2  PowerInvariant=off  UseWithEmbedded=on  PhaseInput=Three inputs
      settings: LibrarySourceBlock=mcbcontrolslib/Clarke Transform
  Demux2 : Demux  Outputs=3
  Gain : Gain  Gain=0.995/sqrt(3)
  Gain1 : Gain  Gain=Psi
  Gain2 : Gain  Gain=PolePairs
  Gain3 : Gain  Gain=FocDiscrTime
  Gain4 : Gain  Gain=Lq
  Gain5 : Gain  Gain=-1
  Gain6 : Gain  Gain=Ld
  Gain7 : Gain  Gain=1-compensate_pwm*0.5
  Inverse Park Transform1 : mcbeeMathTransformLib/Park to Clarke Angle Transform  AxisAlignment=D-axis  UseWithEmbedded=on  PhaseInput=Two inputs  ThetaInput=Electrical position  AngleInput=Radians  N_points=1024
      settings: LibrarySourceBlock=mcbcontrolslib/Inverse Park Transform
  Mux : Mux  Inputs=3
  Mux1 : Mux  Inputs=3
  PID Controller3 : slpidlib/PID Controller  Controller=PI  Form=Parallel  TimeDomain=Discrete-time  UseExternalTs=off  SampleTime=-1  IntegratorMethod=Forward Euler  FilterMethod=Forward Euler  ControllerParametersSource=internal  P=piBandwidth*Ld  I=piBandwidth*Lq  UseKiTs=off  D=0  UseExternalDerivativeSource=off  N=100  UseFilter=on  TunerSelectOption=Transfer Function Based (PID Tuner App)  InitialConditionSource=internal  InitialConditionForIntegrator=0  InitialConditionForFilter=0  DifferentiatorICPrevScaledInput=0  ExternalReset=none  TrackingMode=off  Kt=1  LimitOutput=on  SatLimitsSource=external  UpperSaturationLimit=230  LowerSaturationLimit=-230  LinearizeAsGain=on  AntiWindupMode=clamping  Kb=1  LimitIntegrator=off  UpperIntegratorSaturationLimit=inf  LowerIntegratorSaturationLimit=-inf  POutMin=[]  POutMax=[]  IOutMin=[]  IOutMax=[]  DOutMin=[]  DOutMax=[]  NOutMin=[]  NOutMax=[]  SumOutMin=[]  SumOutMax=[]  SaturationOutMin=[]  SaturationOutMax=[]  PParamMin=[]  PParamMax=[]  IParamMin=[]  IParamMax=[]  DParamMin=[]  DParamMax=[]  NParamMin=[]  NParamMax=[]  KbParamMin=[]  KbParamMax=[]  KtParamMin=[]  KtParamMax=[]  KbOutMin=[]  KbOutMax=[]  KtOutMin=[]  KtOutMax=[]  IntegratorOutMin=[]  IntegratorOutMax=[]  FilterOutMin=[]  FilterOutMax=[]  SumI1OutMin=[]  SumI1OutMax=[]  SumI2OutMin=[]  SumI2OutMax=[]  SumI3OutMin=[]  SumI3OutMax=[]  SumI4OutMin=[]  SumI4OutMax=[]  SumDOutMin=[]  SumDOutMax=[]  DifferentiatorOutMin=[]  DifferentiatorOutMax=[]  FilterDiffOutCoefMin=[]  FilterDiffOutCoefMax=[]  ReciprocalOutMin=[]  ReciprocalOutMax=[]  SumDenOutMin=[]  SumDenOutMax=[]  SumNumOutMin=[]  SumNumOutMax=[]  DivideOutMin=[]  DivideOutMax=[]  UdiffTsProdOutMin=[]  UdiffTsProdOutMax=[]  NTsProdOutMin=[]  NTsProdOutMax=[]  UintegralTsProdOutMin=[]  UintegralTsProdOutMax=[]  UngainTsProdOutMin=[]  UngainTsProdOutMax=[]  ClampingZeroOutDataTypeStr=Inherit: Inherit via back propagation  ClampingZeroOutMin=[]  ClampingZeroOutMax=[]  FilterDenConstantOutDataTypeStr=Inherit: Inherit via back propagation  FilterDenConstantOutMin=[]  FilterDenConstantOutMax=[]  PCopyOutDataTypeStr=Inherit: Inherit via back propagation  PCopyOutMin=[]  PCopyOutMax=[]  NCopyOutDataTypeStr=Inherit: Inherit via back propagation  NCopyOutMin=[]  NCopyOutMax=[]  IntegratorContinuousStateAttributes=''  IntegratorStateMustResolveToSignalObject=off  IntegratorRTWStateStorageClass=Auto  FilterContinuousStateAttributes=''  FilterStateMustResolveToSignalObject=off  FilterRTWStateStorageClass=Auto  ParallelPVariant=InternalParameters  IdealPVariant=Disabled  IVariant=InternalParameters  DVariant=Disabled  IntegratorVariant=Discrete  SatVariant=External  AWVariant=DiscClampingParallel  PCopyVariant=Disabled  TRVariant=Disabled  FdbkBlocksVariant=Forward  IdealPFdbkVariant=Disabled  SatFdbkVariant=Disabled  DerivativeFilterVariant=Disabled  NVariant=Disabled  NCopyVariant=Disabled_SignalSpec  FilterICVariant=Disabled  IntegratorICVariant=InternalICs  ExternalResetVariant=Disabled  TRSumVariant=Passthrough  SumFdbkVariant=Disabled  SumVariant=Sum_PI  TsampFilterVariant=InternalTs  TsampNgainVariant=Passthrough  TsampIntegralVariant=Disabled_SignalSpec  ExternalSaturationOutDataTypeStr=Inherit: Same as second input  DerivativeSourceVariant=Disabled  PreIntVariant=InternalPreInt
  PID Controller4 : slpidlib/PID Controller  Controller=PI  Form=Parallel  TimeDomain=Discrete-time  UseExternalTs=off  SampleTime=-1  IntegratorMethod=Forward Euler  FilterMethod=Forward Euler  ControllerParametersSource=internal  P=piBandwidth*Lq  I=piBandwidth*Rs  UseKiTs=off  D=0  UseExternalDerivativeSource=off  N=100  UseFilter=on  TunerSelectOption=Transfer Function Based (PID Tuner App)  InitialConditionSource=internal  InitialConditionForIntegrator=0  InitialConditionForFilter=0  DifferentiatorICPrevScaledInput=0  ExternalReset=none  TrackingMode=off  Kt=1  LimitOutput=on  SatLimitsSource=external  UpperSaturationLimit=24  LowerSaturationLimit=-15  LinearizeAsGain=on  AntiWindupMode=clamping  Kb=1  LimitIntegrator=off  UpperIntegratorSaturationLimit=inf  LowerIntegratorSaturationLimit=-inf  POutMin=[]  POutMax=[]  IOutMin=[]  IOutMax=[]  DOutMin=[]  DOutMax=[]  NOutMin=[]  NOutMax=[]  SumOutMin=[]  SumOutMax=[]  SaturationOutMin=[]  SaturationOutMax=[]  PParamMin=[]  PParamMax=[]  IParamMin=[]  IParamMax=[]  DParamMin=[]  DParamMax=[]  NParamMin=[]  NParamMax=[]  KbParamMin=[]  KbParamMax=[]  KtParamMin=[]  KtParamMax=[]  KbOutMin=[]  KbOutMax=[]  KtOutMin=[]  KtOutMax=[]  IntegratorOutMin=[]  IntegratorOutMax=[]  FilterOutMin=[]  FilterOutMax=[]  SumI1OutMin=[]  SumI1OutMax=[]  SumI2OutMin=[]  SumI2OutMax=[]  SumI3OutMin=[]  SumI3OutMax=[]  SumI4OutMin=[]  SumI4OutMax=[]  SumDOutMin=[]  SumDOutMax=[]  DifferentiatorOutMin=[]  DifferentiatorOutMax=[]  FilterDiffOutCoefMin=[]  FilterDiffOutCoefMax=[]  ReciprocalOutMin=[]  ReciprocalOutMax=[]  SumDenOutMin=[]  SumDenOutMax=[]  SumNumOutMin=[]  SumNumOutMax=[]  DivideOutMin=[]  DivideOutMax=[]  UdiffTsProdOutMin=[]  UdiffTsProdOutMax=[]  NTsProdOutMin=[]  NTsProdOutMax=[]  UintegralTsProdOutMin=[]  UintegralTsProdOutMax=[]  UngainTsProdOutMin=[]  UngainTsProdOutMax=[]  ClampingZeroOutDataTypeStr=Inherit: Inherit via back propagation  ClampingZeroOutMin=[]  ClampingZeroOutMax=[]  FilterDenConstantOutDataTypeStr=Inherit: Inherit via back propagation  FilterDenConstantOutMin=[]  FilterDenConstantOutMax=[]  PCopyOutDataTypeStr=Inherit: Inherit via back propagation  PCopyOutMin=[]  PCopyOutMax=[]  NCopyOutDataTypeStr=Inherit: Inherit via back propagation  NCopyOutMin=[]  NCopyOutMax=[]  IntegratorContinuousStateAttributes=''  IntegratorStateMustResolveToSignalObject=off  IntegratorRTWStateStorageClass=Auto  FilterContinuousStateAttributes=''  FilterStateMustResolveToSignalObject=off  FilterRTWStateStorageClass=Auto  ParallelPVariant=InternalParameters  IdealPVariant=Disabled  IVariant=InternalParameters  DVariant=Disabled  IntegratorVariant=Discrete  SatVariant=External  AWVariant=DiscClampingParallel  PCopyVariant=Disabled  TRVariant=Disabled  FdbkBlocksVariant=Forward  IdealPFdbkVariant=Disabled  SatFdbkVariant=Disabled  DerivativeFilterVariant=Disabled  NVariant=Disabled  NCopyVariant=Disabled_SignalSpec  FilterICVariant=Disabled  IntegratorICVariant=InternalICs  ExternalResetVariant=Disabled  TRSumVariant=Passthrough  SumFdbkVariant=Disabled  SumVariant=Sum_PI  TsampFilterVariant=InternalTs  TsampNgainVariant=Passthrough  TsampIntegralVariant=Disabled_SignalSpec  ExternalSaturationOutDataTypeStr=Inherit: Same as second input  DerivativeSourceVariant=Disabled  PreIntVariant=InternalPreInt
  Park Transform : mcbeeMathTransformLib/Clarke to Park Angle Transform  AxisAlignment=D-axis  UseWithEmbedded=on  PhaseInput=Two inputs  ThetaInput=Electrical position  AngleInput=Radians  N_points=1024
      settings: LibrarySourceBlock=mcbcontrolslib/Park Transform
  Product : Product
  Product1 : Product
  ScopeComp : Scope  NumInputPorts=3
      settings: ActiveDisplayYMinimum=-69.543787851538823  ActiveDisplayYMaximum=282.10108753848311
  ScopeUd : Scope  NumInputPorts=5
      settings: ActiveDisplayYMinimum=-25.450772374968579  ActiveDisplayYMaximum=2.9110654698893024  DataLoggingVariableName=ScopeData6
  ScopeUq : Scope  NumInputPorts=6
      settings: ActiveDisplayYMinimum=-42.121034586131863  ActiveDisplayYMaximum=354.68011495401464  DataLoggingVariableName=ScopeData4
  Sqrt : Sqrt
  Square : Math  Operator=square
  Square1 : Math  Operator=square
  Sum : Sum  Inputs=-+|
  Sum1 : Sum  Inputs=-+|
  Sum2 : Sum  Inputs=|++
  Sum3 : Sum  Inputs=|++
  Sum4 : Sum
  Sum5 : Sum  Inputs=|++
  Sum6 : Sum  Inputs=-+|
  Sum7 : Sum  Inputs=|+-
  Sum8 : Sum  Inputs=|+-
  Sum9 : Sum  Inputs=++|
  Terminator : Terminator
  Unary Minus1 : UnaryMinus
  UqLimiter : Subsystem
  vRef : Outport
  vAngle : Outport  Port=2
  Vd : Outport  Port=3
  Vq : Outport  Port=4
  Currents_work : Outport  Port=5
  Currents_dq_calc : Outport  Port=6
  Ang : Outport  Port=7
  VDC : Outport  Port=8
  wires:
  Gain/1 -> Sum9/2
  [Uq_lim] -> Sum8/1
  Sum8/1 -> Sum7/1
  [Idreq] -> Sum/2
  Sum6/1 -> [Ud], ScopeUd/4
  speed/1 -> Gain2/1
  angle/1 -> [angle_act], Sum2/1
  Sum2/1 -> [angle_futute]
  currents/1 -> [currents], Clarke Transform/1
  Demux2/1 -> Park Transform/1
  Park Transform/2 -> [Iq]
  Demux2/3 -> Terminator/1
  [Iqreq] -> ScopeUq/1, Sum1/2
  Clarke Transform/1 -> Demux2/1
  Sum/1 -> ScopeUd/2, PID Controller3/1
  Demux2/2 -> Park Transform/2
  Park Transform/1 -> [Id]
  PID Controller4/1 -> ScopeUq/3, Sum5/1
  Sum1/1 -> ScopeUq/2, PID Controller4/1
  Sum5/1 -> Sum3/1
  Unary Minus1/1 -> Mux/2, PID Controller4/3
  Inverse Park Transform1/1 -> Cartesian to Polar1/1
  Inverse Park Transform1/2 -> Cartesian to Polar1/2
  PID Controller3/1 -> Sum6/2, ScopeUd/5
  Mux1/1 -> Currents_dq_calc/1
  [angle_act] -> Park Transform/3
  [angle_futute] -> Inverse Park Transform1/3
  [ElOmega] -> Gain4/1
  Gain4/1 -> Product/2
  Gain6/1 -> Product1/2
  [UdComp] -> Sum6/1, Sum9/1, ScopeUd/1
  [Ecomp] -> Sum8/2, ScopeUq/4, Sum5/2
  [UqComp] -> Sum7/2, Sum3/2, ScopeUq/5
  [Ud] -> UqLimiter/1(In1)
  [VDC] -> UqLimiter/2(In2)
  UqLimiter/1(Out1) -> [Uq_lim]
  Gain2/1 -> [ElOmega], Gain3/1
  Gain3/1 -> Gain7/1
  Gain1/1 -> ScopeComp/1, [Ecomp]
  [ElOmega] -> Gain1/1
  [Id] -> Product1/1
  [Iq] -> Product/1
  [ElOmega] -> Gain6/1
  Product1/1 -> ScopeComp/2, [UqComp]
  Product/1 -> ScopeComp/3, [UdComp]
  [Id] -> Square/1, Mux1/1
  [Iq] -> Square1/1, Mux1/2
  [Ud] -> Vd/1
  [Uq] -> Vq/1
  Sum7/1 -> Unary Minus1/1, Mux/1, PID Controller4/2
  [currents] -> Currents_work/1
  Idreq/1 -> [Idreq]
  Iqreq/1 -> [Iqreq]
  [Ud] -> Inverse Park Transform1/1
  [Uq] -> Inverse Park Transform1/2
  [Id] -> Sum/1
  [Iq] -> Sum1/1
  Vdc/1 -> [VDC]
  [VDC] -> Gain/1
  Sum9/1 -> PID Controller3/2, ScopeUd/3, Gain5/1
  Gain5/1 -> PID Controller3/3
  Gain7/1 -> Sum2/2
  [angle_act] -> Ang/1
  Cartesian to Polar1/2 -> vAngle/1
  Cartesian to Polar1/1 -> vRef/1
  [VDC] -> VDC/1
  Square/1 -> Sum4/1
  Square1/1 -> Sum4/2
  Sum4/1 -> Sqrt/1
  Sqrt/1 -> Mux1/3
  Mux/1 -> ScopeUq/6
  Sum3/1 -> [Uq], Mux/3
